simulink model "aircraft_simulation"  (R2025a)
settings: Solver=ode14x  StartTime=0.0  StopTime=600  FixedStep=0.001  RelTol=1e-3
values from neighbouring files (symbols this model uses):
  c_visc = 0.45    [aircraft_parameters.m]
  k_thrust = 0.05    [aircraft_parameters.m]
  m_aircraft = 3.9    [aircraft_parameters.m]
  V_batt_nom = Ns*V_nom_cell    (= 18.5)    [aircraft_parameters.m]
libraries: fl_lib x6, nesl_utility x4, ee_lib x1
settings Model: Creator=charizardmigo  LastModifiedBy=charizardmigo

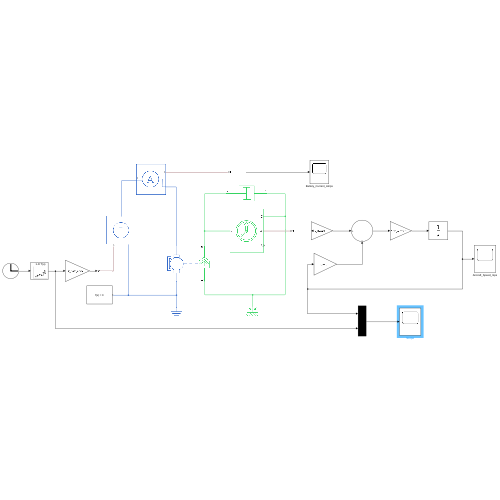
[thumbnail: Simulink's stored preview of the top-level diagram]
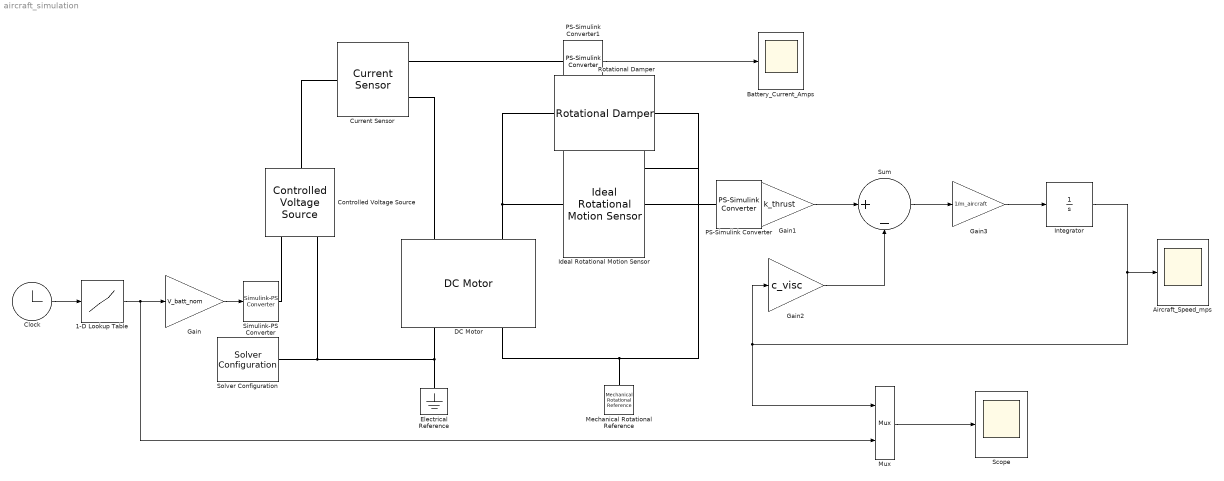
== system aircraft_simulation ==
  1-D Lookup Table : Lookup_n-D  NumberOfTableDimensions=1  BreakpointsForDimension1=[0, 40, 60, 600]  Table=[1.0, 0.5, 0.35, 0.35]  InterpMethod=Flat  InternalRulePriority=Speed  RndMeth=Simplest
  Aircraft_Speed_mps : Scope
      settings: ActiveDisplayYMinimum=0.035366771453870349  ActiveDisplayYMaximum=24.227631055572836
  Battery_Current_Amps : Scope
      settings: ActiveDisplayYMinimum=104.43996153313179  ActiveDisplayYMaximum=385.71552643498029
  Clock : Clock
  Controlled Voltage Source : fl_lib/Electrical/Electrical Sources/Controlled Voltage Source
  Current Sensor : fl_lib/Electrical/Electrical Sensors/Current Sensor
  DC Motor : ee_lib/Electromechanical/Brushed Motors/DC Motor  field_option=ee.enum.field_option.pm  Rf=100 Ohm  Lf=1 H  Laf=0.15 H  If0=0 A  parameterization=ee.enum.dcparam_option.circuit_param  Ra=0.05 Ohm  La=12e-6 H  emf_or_torque=ee.enum.emf_or_torque.kv  Kv=0.072e-3 V/rpm  Ki=6.876e-4 N*m/A  T_stall=0.24e-3 N*m  w_max=19100 rpm  w_rated=15000 rpm  P_rated=0.08 W  V_rated=1.5 V  lam_param=ee.enum.lam_param.damping  i_noload=0 A  V_i_noload=1.5 V  J=0.01 cm^2*g  lam=0 N*m*s/rad  speed0=0 rpm  alpha=3.93e-3 1/K  Tmeas=25 degC  thermal_mass=100 J/K  initial_temperature=25 degC
  Electrical Reference : fl_lib/Electrical/Electrical Elements/Electrical Reference
  Gain : Gain  Gain=V_batt_nom
  Gain1 : Gain  Gain=k_thrust
  Gain2 : Gain  Gain=c_visc
  Gain3 : Gain  Gain=1/m_aircraft
  Ideal Rotational Motion Sensor : fl_lib/Mechanical/Mechanical Sensors/Ideal Rotational Motion Sensor  reference=foundation.enum.MeasurementReference.difference  acceleration_port=false  velocity_port=true  position_port=true  wrap_angle=false  offset=0 rad
  Integrator : Integrator
  Mechanical Rotational Reference : fl_lib/Mechanical/Rotational Elements/Mechanical Rotational Reference
  Mux : Mux  Inputs=2
  PS-Simulink Converter : nesl_utility/PS-Simulink Converter  PhysicalDomain=network_engine_domain  SubClassName=ps_output  LeftPortType=input  RightPortType=output  PseudoPeriodic=off  Frequencies=[]  VectorFormat=inherit  Unit=inherit  AffineConversion=off
  PS-Simulink Converter1 : nesl_utility/PS-Simulink Converter  PhysicalDomain=network_engine_domain  SubClassName=ps_output  LeftPortType=input  RightPortType=output  PseudoPeriodic=off  Frequencies=[]  VectorFormat=inherit  Unit=inherit  AffineConversion=off
  Rotational Damper : fl_lib/Mechanical/Rotational Elements/Rotational Damper  D=0.001 N*m*s/rad  w_specify=off  w_priority=None  w=0 rad/s  w_nominal_specify=off  w_nominal_value=1  w_nominal_unit=rad/s  t_specify=off  t_priority=None  t=0 N*m  t_nominal_specify=off  t_nominal_value=1  t_nominal_unit=N*m
  Scope : Scope
      settings: ActiveDisplayYMinimum=0.26754220900700654  ActiveDisplayYMaximum=1.0619750471960434  DataLoggingVariableName=ScopeData2
  Simulink-PS Converter : nesl_utility/Simulink-PS Converter  PhysicalDomain=network_engine_domain  SubClassName=ps_input  LeftPortType=input  RightPortType=output  PseudoPeriodic=off  Frequencies=[]  NoiseDistribution=none  NoiseParameters=[]  Unit=V  AffineConversion=off  FilteringAndDerivatives=provide  SimscapeFilterOrder=1  InputFilterTimeConstant=0.001  UdotUserProvided=0
  Solver Configuration : nesl_utility/Solver Configuration  PhysicalDomain=network_engine_domain  SubClassName=solver  LeftPortType=input  RightPortType=generic  Tones=[]  Harmonics=[]  SimulateNoise=off  Profile=off  UseLocalSampling=off  EnableSwitchedLinearOptims=on  FrequencyDomain=off  UseCCode=off  RelTol=0.001  AbsTol=0.001  MinStep=1e-09  ToWorkspace=off  RevertToSquareIcSolve=off  NumHomotopyIterations=100  PhasorMode=off  PhasorModeNumHarmonics=1  ConsistencySolver=NEWTON_XTOL_AFTER_FTOL  IndexReductionMethod=DerivativeReplacement  DoDC=off  ResidualTolerance=1e-09  ConsistencyTolSource=GLOBAL  ConsistencyAbsTol=0.001  ConsistencyRelTol=0.001  ConsistencyTolFactor=0.001  UseLocalSolver=off  LocalSolverChoice=NE_BACKWARD_EULER_ADVANCER  ResolveIndetEquations=on  FunctionEvalNumThread=1  LocalSolverSampleTime=0.001  DoFixedCost=off  MaxNonlinIter=3  MaxModeIter=2  ComputeImpulses=off  ImpulseIterations=2  LinearAlgebra=auto  LinearAlgebraNumThread=0  EquationFormulation=NE_TIME_EF  DelaysMemoryBudget=1024  AutomaticFiltering=on  FilteringTimeConstant=0.001  PartitionStorageMethod=AS_NEEDED  PartitionMemoryBudget=1024  PartitionMethod=ROBUST  MultibodyUseLocalSolver=off  MultibodyLocalSolverChoice=ODE1  MultibodyLocalSolverSampleTime=0.001
  Sum : Sum  Inputs=|+-
  wires:
  Clock/1 -> 1-D Lookup Table/1
  1-D Lookup Table/1 -> Mux/2, Gain/1
  Gain/1 -> Simulink-PS Converter/1
  PS-Simulink Converter/1 -> Gain1/1
  Gain2/1 -> Sum/2
  Gain3/1 -> Integrator/1
  Integrator/1 -> Mux/1, Gain2/1, Aircraft_Speed_mps/1
  PS-Simulink Converter1/1 -> Battery_Current_Amps/1
  Mux/1 -> Scope/1
  Sum/1 -> Gain3/1
  Gain1/1 -> Sum/1
  connections:
  Controlled Voltage Source/RConn2 -- Electrical Reference/LConn1 -- DC Motor/RConn1 -- Solver Configuration/RConn1
  Controlled Voltage Source/RConn1 -- Simulink-PS Converter/RConn1
  Mechanical Rotational Reference/LConn1 -- Rotational Damper/RConn1 -- Ideal Rotational Motion Sensor/RConn1 -- DC Motor/RConn2
  Rotational Damper/LConn1 -- Ideal Rotational Motion Sensor/LConn1 -- DC Motor/LConn2
  Ideal Rotational Motion Sensor/RConn2 -- PS-Simulink Converter/LConn1
  Controlled Voltage Source/LConn1 -- Current Sensor/LConn1
  PS-Simulink Converter1/LConn1 -- Current Sensor/RConn1
  Current Sensor/RConn2 -- DC Motor/LConn1
